simulink model "s_b4a4x32kf_nb"  (R2018a)
settings: Solver=VariableStepDiscrete  StartTime=0.0  StopTime=10000  RelTol=1e-3
undefined symbols (not defined in the file): fft_stages, n_bits_ants, n_bits_xengs
libraries: xbsIndex_r4 x21193, casper_library_misc x37, casper_library_scopes x13, casper_library_delays x8, xbsReplacements_r4 x6, xps_library x4
(part 98 of 274)

== system s_b4a4x32kf_nb/sys2/pkt_reord/Subsystem7 ==
  dv : Inport
  Constant8 : xbsIndex_r4/Constant  const=clk_rate  gui_display_data_type=Fixed-point  arith_type=Unsigned  n_bits=ceil(log2(clk_rate))  bin_pt=0  preci_type=Single  exp_width=8  frac_width=24  explicit_period=on  period=1  equ=P=C  opselect=C  inp2=PCIN>>17  opr=+  inp1=P  carry=CIN  dbl_ovrd=off  block_type=constant
      settings: SourceProductName=The database /home/jmanley/.matlab/R2018a/slblocks_master.db is locked, or a table in the database is locked. (database is locked)  block_version=11.4
  Counter1 : xbsIndex_r4/Counter  cnt_type=Count Limited  cnt_to=clk_rate  operation=Up  start_count=0  cnt_by_val=1  arith_type=Unsigned  n_bits=ceil(log2(clk_rate))  bin_pt=0  load_pin=off  rst=off  en=off  explicit_period=on  period=1  use_behavioral_HDL=off  implementation=Fabric  dbl_ovrd=off  block_type=counter
      settings: SourceProductName=The database /home/jmanley/.matlab/R2018a/slblocks_master.db is locked, or a table in the database is locked. (database is locked)
  Counter6 : xbsIndex_r4/Counter  cnt_type=Free Running  cnt_to=Inf  operation=Up  start_count=0  cnt_by_val=1  arith_type=Unsigned  n_bits=32  bin_pt=0  load_pin=off  rst=on  en=on  explicit_period=on  period=1  use_behavioral_HDL=off  implementation=Fabric  dbl_ovrd=off  block_type=counter
      settings: SourceProductName=The database /home/jmanley/.matlab/R2018a/slblocks_master.db is locked, or a table in the database is locked. (database is locked)
  Delay : xbsIndex_r4/Delay  rst=off  infoeditControl=Selection of Reset will increase slice count due to use of real FFs and instead of SRLs  en=on  latency=1  reg_retiming=on  dbl_ovrd=off  block_type=delay
      settings: SourceProductName=The database /home/jmanley/.matlab/R2018a/slblocks_master.db is locked, or a table in the database is locked. (database is locked)  infoedit=Hardware notes: A delay line is a chain, each link of which is an SRL16 or SRL32 followed by a flip-flop.
  Delay5 : xbsIndex_r4/Delay  rst=off  infoeditControl=Selection of Reset will increase slice count due to use of real FFs and instead of SRLs  en=off  latency=1  reg_retiming=on  dbl_ovrd=off  block_type=delay
      settings: SourceProductName=The database /home/jmanley/.matlab/R2018a/slblocks_master.db is locked, or a table in the database is locked. (database is locked)  infoedit=Hardware notes: A delay line is a chain, each link of which is an SRL16 or SRL32 followed by a flip-flop.
  Relational : xbsIndex_r4/Relational  mode=a=b  op_type=Bool  en=off  latency=1  dbl_ovrd=off  block_type=relational
      settings: SourceProductName=The database /home/jmanley/.matlab/R2018a/slblocks_master.db is locked, or a table in the database is locked. (database is locked)
  per_sec : Outport
  wires:
  Delay/1 -> per_sec/1
  Counter6/1 -> Delay/1
  dv/1 -> Delay5/1
  Relational/1 -> Delay/2, Counter6/1
  Counter1/1 -> Relational/1
  Delay5/1 -> Counter6/2
  Constant8/1 -> Relational/2

== system s_b4a4x32kf_nb/sys2/pkt_reord/bus_expand ==
  bus_in : Inport
  reinterpret1 : xbsIndex_r4/Reinterpret  force_arith_type=on  arith_type=Unsigned  force_bin_pt=on  bin_pt=0  block_type=reinterpret
      settings: SourceProductName=The database /home/jmanley/.matlab/R2018a/slblocks_master.db is locked, or a table in the database is locked. (database is locked)
  slice1 : xbsIndex_r4/Slice  nbits=32  boolean_output=off  mode=Upper Bit Location + Width  bit1=-1  base1=MSB of Input  bit0=0  base0=LSB of Input  dbl_ovrd=off  block_type=slice
      settings: SourceProductName=The database /home/jmanley/.matlab/R2018a/slblocks_master.db is locked, or a table in the database is locked. (database is locked)
  slice2 : xbsIndex_r4/Slice  nbits=1  boolean_output=on  mode=Upper Bit Location + Width  bit1=0  base1=MSB of Input  bit0=0  base0=LSB of Input  dbl_ovrd=off  block_type=slice
      settings: SourceProductName=The database /home/jmanley/.matlab/R2018a/slblocks_master.db is locked, or a table in the database is locked. (database is locked)
  msb_out2 : Outport
  lsb_out1 : Outport  Port=2
  wires:
  bus_in/1 -> slice2/1, slice1/1
  slice2/1 -> msb_out2/1
  slice1/1 -> reinterpret1/1
  reinterpret1/1 -> lsb_out1/1

== system s_b4a4x32kf_nb/sys2/pkt_reord/bus_replicate ==
  in : Inport
  bussify : Subsystem  mask(bus_create){inputNum=1}
      mask prompts: inputNum "Number of inputs:"
      mask init:
      | bus_create_init(gcb,...
      |     'inputNum', inputNum);
  out : Outport
  wires:
  in/1 -> bussify/1(in1)
  bussify/1(bus_out) -> out/1

== system s_b4a4x32kf_nb/sys2/pkt_reord/input_control ==
  note: Allow writing to windows
      | up to 1/2 the total buffer size
      |  behind the current maximum
      | mcnt
  data_in : Inport
  valid : Inport  Port=2
  pkt_idx : Inport  Port=3
  time_freq : Inport  Port=4
  src : Inport  Port=5
  pkt_size : Inport  Port=6
  n_src : Inport  Port=7
  AddSub2 : xbsIndex_r4/AddSub  mode=Addition  use_carryin=off  use_carryout=off  en=off  latency=2  precision=User Defined  arith_type=Unsigned  n_bits=n_bits_timestamp+chan_bits-xeng_bits  bin_pt=0  quantization=Truncate  overflow=Wrap  use_behavioral_HDL=on  hw_selection=Fabric  pipelined=off  use_rpm=on  dbl_ovrd=off  block_type=addsub
      settings: SourceProductName=The database /home/jmanley/.matlab/R2018a/slblocks_master.db is locked, or a table in the database is locked. (database is locked)  xl_area=[0, 0, 0, 0, 0, 0, 0]  block_version=10.1.3
  Constant2 : xbsIndex_r4/Constant  const=2^(window_bits - 1)  gui_display_data_type=Fixed-point  arith_type=Unsigned  n_bits=n_bits_timestamp+chan_bits-xeng_bits  bin_pt=0  preci_type=Single  exp_width=8  frac_width=24  explicit_period=on  period=1  equ=P=C  opselect=C  inp2=PCIN>>17  opr=+  inp1=P  carry=CIN  dbl_ovrd=off  block_type=constant
      settings: SourceProductName=The database /home/jmanley/.matlab/R2018a/slblocks_master.db is locked, or a table in the database is locked. (database is locked)
  Constant4 : xbsIndex_r4/Constant  const=0  gui_display_data_type=Boolean  arith_type=Boolean  n_bits=16  bin_pt=14  preci_type=Single  exp_width=8  frac_width=24  explicit_period=on  period=1  equ=P=C  opselect=C  inp2=PCIN>>17  opr=+  inp1=P  carry=CIN  dbl_ovrd=off  block_type=constant
      settings: SourceProductName=The database /home/jmanley/.matlab/R2018a/slblocks_master.db is locked, or a table in the database is locked. (database is locked)  block_version=11.4
  Delay{11,13..14,16} (4 alike) : xbsIndex_r4/Delay  rst=off  infoeditControl=Selection of Reset will increase slice count due to use of real FFs and instead of SRLs  en=off  latency=1  reg_retiming=on  dbl_ovrd=off  block_type=delay
      settings: SourceProductName=The database /home/jmanley/.matlab/R2018a/slblocks_master.db is locked, or a table in the database is locked. (database is locked)  infoedit=Hardware notes: A delay line is a chain, each link of which is an SRL16 or SRL32 followed by a flip-flop.  xl_area=[0, 0, 0, 0, 0, 0, 0]
  Delay{2,4..5,8..9} (5 alike) : xbsIndex_r4/Delay  rst=off  infoeditControl=Selection of Reset will increase slice count due to use of real FFs and instead of SRLs  en=off  latency=2  reg_retiming=on  dbl_ovrd=off  block_type=delay
      settings: SourceProductName=The database /home/jmanley/.matlab/R2018a/slblocks_master.db is locked, or a table in the database is locked. (database is locked)  xl_area=[0, 0, 0, 0, 0, 0, 0]
  Delay{3,21,24..27} (6 alike) : xbsIndex_r4/Delay  rst=off  infoeditControl=Selection of Reset will increase slice count due to use of real FFs and instead of SRLs  en=off  latency=3  reg_retiming=on  dbl_ovrd=off  block_type=delay
      settings: SourceProductName=The database /home/jmanley/.matlab/R2018a/slblocks_master.db is locked, or a table in the database is locked. (database is locked)  xl_area=[0, 0, 0, 0, 0, 0, 0]
  Delay23 : xbsIndex_r4/Delay  rst=off  infoeditControl=Selection of Reset will increase slice count due to use of real FFs and instead of SRLs  en=off  latency=4  reg_retiming=on  dbl_ovrd=off  block_type=delay
      settings: SourceProductName=The database /home/jmanley/.matlab/R2018a/slblocks_master.db is locked, or a table in the database is locked. (database is locked)  xl_area=[0, 0, 0, 0, 0, 0, 0]
  Inverter : xbsIndex_r4/Inverter  en=off  latency=0  dbl_ovrd=off  block_type=inv
      settings: SourceProductName=The database /home/jmanley/.matlab/R2018a/slblocks_master.db is locked, or a table in the database is locked. (database is locked)
  Logical : xbsIndex_r4/Logical  logical_function=AND  inputs=3  en=off  latency=1  precision=Full  arith_type=Unsigned  n_bits=8  bin_pt=2  align_bp=on  dbl_ovrd=off  block_type=logical
      settings: SourceProductName=The database /home/jmanley/.matlab/R2018a/slblocks_master.db is locked, or a table in the database is locked. (database is locked)  xl_area=[0, 0, 0, 0, 0, 0, 0]
  Logical1 : xbsIndex_r4/Logical  logical_function=AND  inputs=2  en=off  latency=0  precision=Full  arith_type=Unsigned  n_bits=8  bin_pt=2  align_bp=on  dbl_ovrd=off  block_type=logical
      settings: SourceProductName=The database /home/jmanley/.matlab/R2018a/slblocks_master.db is locked, or a table in the database is locked. (database is locked)  xl_area=[0, 0, 0, 0, 0, 0, 0]
  Mult : xbsIndex_r4/Mult  precision=Full  arith_type=Unsigned  n_bits=buf_bits  bin_pt=0  quantization=Truncate  overflow=Wrap  en=off  latency=3  use_behavioral_HDL=off  opt=Speed  use_embedded=on  optimum_pipeline=off  pipeline=on  dbl_ovrd=off  use_rpm=on  placement_style=Triangular  block_type=mult
      settings: SourceProductName=The database /home/jmanley/.matlab/R2018a/slblocks_master.db is locked, or a table in the database is locked. (database is locked)
  Mult1 : xbsIndex_r4/Mult  precision=Full  arith_type=Unsigned  n_bits=buf_bits  bin_pt=0  quantization=Truncate  overflow=Wrap  en=off  latency=3  use_behavioral_HDL=off  opt=Speed  use_embedded=on  optimum_pipeline=off  pipeline=on  dbl_ovrd=off  use_rpm=on  placement_style=Triangular  block_type=mult
      settings: SourceProductName=The database /home/jmanley/.matlab/R2018a/slblocks_master.db is locked, or a table in the database is locked. (database is locked)
  Relational : xbsIndex_r4/Relational  mode=a>=b  op_type=Bool  en=off  latency=2  dbl_ovrd=off  block_type=relational
      settings: SourceProductName=The database /home/jmanley/.matlab/R2018a/slblocks_master.db is locked, or a table in the database is locked. (database is locked)  xl_area=[0, 0, 0, 0, 0, 0, 0]  block_version=10.1.3
  Relational2 : xbsIndex_r4/Relational  mode=a<b  op_type=Bool  en=off  latency=2  dbl_ovrd=off  block_type=relational
      settings: SourceProductName=The database /home/jmanley/.matlab/R2018a/slblocks_master.db is locked, or a table in the database is locked. (database is locked)  xl_area=[0, 0, 0, 0, 0, 0, 0]  block_version=10.1.3
  Slice1 : xbsIndex_r4/Slice  nbits=buf_bits  boolean_output=off  mode=Lower Bit Location + Width  bit1=0  base1=MSB of Input  bit0=0  base0=LSB of Input  dbl_ovrd=off  block_type=slice
      settings: SourceProductName=The database /home/jmanley/.matlab/R2018a/slblocks_master.db is locked, or a table in the database is locked. (database is locked)
  Slice2 : xbsIndex_r4/Slice  nbits=window_bits  boolean_output=off  mode=Lower Bit Location + Width  bit1=0  base1=MSB of Input  bit0=0  base0=LSB of Input  dbl_ovrd=off  block_type=slice
      settings: SourceProductName=The database /home/jmanley/.matlab/R2018a/slblocks_master.db is locked, or a table in the database is locked. (database is locked)
  Terminator : Terminator
  adder_tree : Subsystem  Tag=cmac_delinked  mask(adder_tree){n_inputs=3, csp_latency=2, adder_imp=Fabric, first_stage_hdl=off, floating_point=off, float_type=single, frac_width=0, exp_width=0}
      mask prompts: n_inputs "Number of Inputs"; csp_latency "Add Latency"; adder_imp "Adder implementation"; first_stage_hdl "Use behavioural HDL for first stage of adders"; floating_point "floating point"; float_type "float type"; frac_width "fraction length"; exp_width "exponent length"
      mask help:
      | Sums all inputs using a tree of adds and delays.
      |
      | Number of inputs: The number of inputs to the block to be summed
      | Add latency: The number of clock cycles to perform one addition (affects timing)..
      | Adder implementation: choice of fabric or DSP48E core, or behavioral HDL
      | Use behavioural HDL for first stage of adders: Causes the first stage of adders to be absorbed into DSP blocks if multipliers precede them (Virtex 5). Overrides Adder implementation
      mask init: same as s_b4a4x32kf_nb/sys0/pkt_reord/input_control/adder_tree
      settings: AttributesFormatString=latency 4
      mask Help: eval('xlWeb(''http://casper.berkeley.edu/wiki/Adder_tree'')')
      mask TypeOptions adder_imp: Behavioral | Fabric | DSP48
      mask Callback floating_point:
      | onoff = get_param(gcb, 'floating_point');
      | if strcmp(onoff,'on')
      |     enable_fixpt = 'off'
      |     set_param_state(gcb, 'float_type', 'on')
      | 
      |     f_type = get_param(gcb, 'float_type')
      |     if strcmp(f_type,'custom')
      |         set_param_state(gcb, 'exp_width', 'on')
      |         set_param_state(gcb, 'frac_width', 'on')
      |     else
      |         set_param_state(gcb, 'exp_width', 'off')
      |         set_param_state(gcb, 'frac_width', 'off')
      |     end
      | 
      | 
      | else
      |     enable_fixpt = 'on'
      |     set_param_state(gcb, 'float_type', 'off')
      |     set_param_state(gcb, 'exp_width', 'off')
      |     set_param_state(gcb, 'frac_width', 'off')
      | end
      mask TypeOptions float_type: single | custom
      mask Callback float_type:
      | f_type = get_param(gcb, 'float_type')
      | if strcmp(f_type,'custom')
      |     set_param_state(gcb, 'exp_width', 'on')
      |     set_param_state(gcb, 'frac_width', 'on')
      | else
      |     set_param_state(gcb, 'exp_width', 'off')
      |     set_param_state(gcb, 'frac_width', 'off')
      | end
  freq_window : xbsIndex_r4/Mult  precision=Full  arith_type="Signed  (2's comp)"  n_bits=16  bin_pt=14  quantization=Truncate  overflow=Wrap  en=off  latency=3  use_behavioral_HDL=off  opt=Speed  use_embedded=on  optimum_pipeline=off  pipeline=on  dbl_ovrd=off  use_rpm=on  placement_style=Triangular  block_type=mult
      settings: SourceProductName=The database /home/jmanley/.matlab/R2018a/slblocks_master.db is locked, or a table in the database is locked. (database is locked)
  mcnt_thresh : Subsystem
  maxcnt : Outport
  wr_addr : Outport  Port=2
  wr_data : Outport  Port=3
  we : Outport  Port=4
  discarding : Outport  Port=5
  mcnt_timeout : Outport  Port=6
  wires:
  Constant2/1 -> AddSub2/2
  Delay2/1 -> Delay4/1
  Delay3/1 -> Delay2/1, [data_add]
  data_in/1 -> Delay3/1
  adder_tree/2(dout) -> Slice1/1
  Slice2/1 -> Mult1/2
  freq_window/1 -> Mult1/1
  n_src/1 -> freq_window/1
  Mult1/1 -> adder_tree/2(din1), [brds_pkt_size_time]
  Delay27/1 -> AddSub2/1
  Delay26/1 -> mcnt_thresh/1(mcnt)
  Delay25/1 -> Delay5/1
  Constant4/1 -> adder_tree/1(sync)
  Mult/1 -> adder_tree/3(din2), [src_pkt_size]
  Delay21/1 -> [pkt_idx], adder_tree/4(din3)
  time_freq/1 -> Slice2/1, Delay26/1, Delay25/1, [mcnt_in], Delay27/1
  Delay24/1 -> mcnt_thresh/2(en), [valid_add], Delay23/1
  src/1 -> Mult/1
  pkt_size/1 -> freq_window/2, Mult/2
  pkt_idx/1 -> Delay21/1
  valid/1 -> Delay24/1
  Delay9/1 -> Delay13/1
  Slice1/1 -> Delay16/1
  Delay4/1 -> Delay11/1
  Delay23/1 -> Logical/3, Delay14/1
  Logical/1 -> Inverter/1, [we], we/1
  Relational/1 -> Logical/2
  Delay5/1 -> Relational/2
  mcnt_thresh/1(maxcnt) -> Delay9/1, Relational2/1, Relational/1
  Relational2/1 -> Logical/1
  adder_tree/1(sync_out) -> Terminator/1
  Logical1/1 -> [discarding], discarding/1
  Inverter/1 -> Logical1/1
  mcnt_thresh/2(mcnt_timeout) -> [timeout], Delay8/1
  AddSub2/1 -> Relational2/2
  Delay11/1 -> wr_data/1, [wr_data]
  Delay13/1 -> maxcnt/1, [max_mcnt]
  Delay14/1 -> Logical1/2
  Delay8/1 -> mcnt_timeout/1
  Delay16/1 -> [wr_addr], wr_addr/1

== system s_b4a4x32kf_nb/sys2/pkt_reord/munge ==
  din : Inport
  join : Subsystem  mask(bus_create){inputNum=16}
      mask prompts: inputNum "Number of inputs:"
      mask init:
      | bus_create_init(gcb,...
      |     'inputNum', inputNum);
  reinterpret : xbsIndex_r4/Reinterpret  force_arith_type=on  arith_type=Unsigned  force_bin_pt=on  bin_pt=0  block_type=reinterpret
      settings: SourceProductName=The database /home/jmanley/.matlab/R2018a/slblocks_master.db is locked, or a table in the database is locked. (database is locked)
  reinterpret_out : xbsIndex_r4/Reinterpret  force_arith_type=on  arith_type=Unsigned  force_bin_pt=on  bin_pt=0  block_type=reinterpret
      settings: SourceProductName=The database /home/jmanley/.matlab/R2018a/slblocks_master.db is locked, or a table in the database is locked. (database is locked)
  split : Subsystem  mask(bus_expand){mode=divisions of arbitrary size, outputNum=1, outputWidth=[1 32 32 32 32 32 32 32 32], outputBinaryPt=[0 0 0 0 0 0 0 0 0], outputArithmeticType=[0 0 0 0 0 0 0 0 0], show_format=off, outputToWorkspace=off, variablePrefix=out, outputToModelAsWell=on}
      mask prompts: outputNum "Number of outputs:"; outputWidth "Output width [msb ... lsb]:"; outputBinaryPt "Output binary point position [msb ... lsb]:"; outputArithmeticType "Output arithmetic type (ufix=0, fix=1, bool=2) [msb ... lsb]:"; show_format "Print format string?"; outputToWorkspace "Output to workspace?"; variablePrefix "Variable name prefix:"; outputToModelAsWell "Output to model as well?"
      mask help:
      | Expands a 'bus' made using a bus_create or Xilinx
      | concat block.
      | The input will be divided into the specified number
      | of outputs with the specified arithmetic types.
      | Divisions are made from most significant bit.
      mask init: same as s_b4a4x32kf_nb/bus_expand
      settings: AttributesFormatString=9 outputs
      mask TypeOptions mode: divisions of equal size | divisions of arbitrary size
      mask Callback mode: bus_expand_callback();
      mask Callback outputWidth: bus_expand_callback();
      mask Callback outputToWorkspace: bus_expand_callback();
  dout : Outport
  wires:
  reinterpret_out/1 -> dout/1
  din/1 -> reinterpret/1
  reinterpret/1 -> split/1(bus_in)
  join/1(bus_out) -> reinterpret_out/1
  split/1(msb_out9) -> join/1(in1), join/3(in3), join/5(in5), join/7(in7), join/9(in9), join/11(in11), join/13(in13), join/15(in15)
  split/9(lsb_out1) -> join/2(in2)
  split/8(out2) -> join/4(in4)
  split/7(out3) -> join/6(in6)
  split/6(out4) -> join/8(in8)
  split/5(out5) -> join/10(in10)
  split/4(out6) -> join/12(in12)
  split/3(out7) -> join/14(in14)
  split/2(out8) -> join/16(in16)

== system s_b4a4x32kf_nb/sys2/pkt_reord/munge1 ==
  din : Inport
  join : Subsystem  mask(bus_create){inputNum=2}
      mask prompts: inputNum "Number of inputs:"
      mask init:
      | bus_create_init(gcb,...
      |     'inputNum', inputNum);
  reinterpret : xbsIndex_r4/Reinterpret  force_arith_type=on  arith_type=Unsigned  force_bin_pt=on  bin_pt=0  block_type=reinterpret
      settings: SourceProductName=The database /home/jmanley/.matlab/R2018a/slblocks_master.db is locked, or a table in the database is locked. (database is locked)
  reinterpret_out : xbsIndex_r4/Reinterpret  force_arith_type=on  arith_type=Unsigned  force_bin_pt=on  bin_pt=0  block_type=reinterpret
      settings: SourceProductName=The database /home/jmanley/.matlab/R2018a/slblocks_master.db is locked, or a table in the database is locked. (database is locked)
  split : Subsystem  mask(bus_expand){mode=divisions of arbitrary size, outputNum=1, outputWidth=[1 32], outputBinaryPt=[0 0], outputArithmeticType=[0 0], show_format=off, outputToWorkspace=off, variablePrefix=out, outputToModelAsWell=on}
      mask prompts: outputNum "Number of outputs:"; outputWidth "Output width [msb ... lsb]:"; outputBinaryPt "Output binary point position [msb ... lsb]:"; outputArithmeticType "Output arithmetic type (ufix=0, fix=1, bool=2) [msb ... lsb]:"; show_format "Print format string?"; outputToWorkspace "Output to workspace?"; variablePrefix "Variable name prefix:"; outputToModelAsWell "Output to model as well?"
      mask help:
      | Expands a 'bus' made using a bus_create or Xilinx
      | concat block.
      | The input will be divided into the specified number
      | of outputs with the specified arithmetic types.
      | Divisions are made from most significant bit.
      mask init: same as s_b4a4x32kf_nb/bus_expand
      settings: AttributesFormatString=2 outputs
      mask TypeOptions mode: divisions of equal size | divisions of arbitrary size
      mask Callback mode: bus_expand_callback();
      mask Callback outputWidth: bus_expand_callback();
      mask Callback outputToWorkspace: bus_expand_callback();
  dout : Outport
  wires:
  reinterpret_out/1 -> dout/1
  din/1 -> reinterpret/1
  reinterpret/1 -> split/1(bus_in)
  join/1(bus_out) -> reinterpret_out/1
  split/1(msb_out2) -> join/1(in1)
  split/2(lsb_out1) -> join/2(in2)

== system s_b4a4x32kf_nb/sys2/pkt_reord/output_control ==
  note: add delay here
      | to ensure mcnt has had
      | chance to calculate
      | correctly
  note: If reading from addr 0 (corresponding to f=0,nant,2nant,...)
      | and max_mcnt (skipping window_bits for the difference
      | between max_mcnt and rd_mcnt) is 0 for sync_bits, then
      | issue a sync.
  note: If we need to ship a window,
      | send the data on a window edge
  note: Decide whether to ship
      | a window or not:
  note: If the read window is 1/2
      | the total buffer size (or more)
      | behind the write window,
      | it is time to ship it out.
  note: rd_addr is counting for
      | output words to
      | X engines
  maxcnt : Inport
  AddSub1 : xbsIndex_r4/AddSub  mode=Subtraction  use_carryin=off  use_carryout=off  en=off  latency=2  precision=User Defined  arith_type=Unsigned  n_bits=window_bits  bin_pt=0  quantization=Truncate  overflow=Wrap  use_behavioral_HDL=on  hw_selection=Fabric  pipelined=off  use_rpm=on  dbl_ovrd=off  block_type=addsub
      settings: SourceProductName=The database /home/jmanley/.matlab/R2018a/slblocks_master.db is locked, or a table in the database is locked. (database is locked)  xl_area=[0, 0, 0, 0, 0, 0, 0]  block_version=10.1.3
  Concat1 : xbsIndex_r4/Concat  num_inputs=2  dbl_ovrd=off  block_type=concat
      settings: SourceProductName=The database /home/jmanley/.matlab/R2018a/slblocks_master.db is locked, or a table in the database is locked. (database is locked)  block_version=10.1.3
  Concat2 : xbsIndex_r4/Concat  num_inputs=2  dbl_ovrd=off  block_type=concat
      settings: SourceProductName=The database /home/jmanley/.matlab/R2018a/slblocks_master.db is locked, or a table in the database is locked. (database is locked)  block_version=10.1.3
  Constant1 : xbsIndex_r4/Constant  const=2^(window_bits - 1)  gui_display_data_type=Fixed-point  arith_type=Unsigned  n_bits=window_bits  bin_pt=0  preci_type=Single  exp_width=8  frac_width=24  explicit_period=on  period=1  equ=P=C  opselect=C  inp2=PCIN>>17  opr=+  inp1=P  carry=CIN  dbl_ovrd=off  block_type=constant
      settings: SourceProductName=The database /home/jmanley/.matlab/R2018a/slblocks_master.db is locked, or a table in the database is locked. (database is locked)
  Constant3 : xbsIndex_r4/Constant  const=0  gui_display_data_type=Fixed-point  arith_type=Unsigned  n_bits=sync_bits - x_int_bits - ant_bits - window_bits  bin_pt=0  preci_type=Single  exp_width=8  frac_width=24  explicit_period=on  period=1  equ=P=C  opselect=C  inp2=PCIN>>17  opr=+  inp1=P  carry=CIN  dbl_ovrd=off  block_type=constant
      settings: SourceProductName=The database /home/jmanley/.matlab/R2018a/slblocks_master.db is locked, or a table in the database is locked. (database is locked)
  Delay1 : xbsIndex_r4/Delay  rst=off  infoeditControl=Selection of Reset will increase slice count due to use of real FFs and instead of SRLs  en=off  latency=1  reg_retiming=on  dbl_ovrd=off  block_type=delay
      settings: SourceProductName=The database /home/jmanley/.matlab/R2018a/slblocks_master.db is locked, or a table in the database is locked. (database is locked)  xl_area=[0, 0, 0, 0, 0, 0, 0]
  Delay3 : xbsIndex_r4/Delay  rst=off  infoeditControl=Selection of Reset will increase slice count due to use of real FFs and instead of SRLs  en=off  latency=2  reg_retiming=on  dbl_ovrd=off  block_type=delay
      settings: SourceProductName=The database /home/jmanley/.matlab/R2018a/slblocks_master.db is locked, or a table in the database is locked. (database is locked)  xl_area=[0, 0, 0, 0, 0, 0, 0]
  Delay6 : xbsIndex_r4/Delay  rst=off  infoeditControl=Selection of Reset will increase slice count due to use of real FFs and instead of SRLs  en=off  latency=1  reg_retiming=on  dbl_ovrd=off  block_type=delay
      settings: SourceProductName=The database /home/jmanley/.matlab/R2018a/slblocks_master.db is locked, or a table in the database is locked. (database is locked)  xl_area=[0, 0, 0, 0, 0, 0, 0]
  Delay7 : xbsIndex_r4/Delay  rst=off  infoeditControl=Selection of Reset will increase slice count due to use of real FFs and instead of SRLs  en=off  latency=2  reg_retiming=on  dbl_ovrd=off  block_type=delay
      settings: SourceProductName=The database /home/jmanley/.matlab/R2018a/slblocks_master.db is locked, or a table in the database is locked. (database is locked)  xl_area=[0, 0, 0, 0, 0, 0, 0]
  Gateway Out{1..18} (18 alike) : xbsIndex_r4/Gateway Out  inherit_from_input=off  hdl_port=off  rows=1  columns=1  UseAsDAC=off  DACChannel='1'  interface=None  automatic_assignment=on  address_offset=hex2dec('00')  intf_name=''  intf_description=''  timing_constraint=None  locs_specified=off  LOCs={}  io_standard={}  block_type=gatewayout
      settings: SourceProductName=The database /home/jmanley/.matlab/R2018a/slblocks_master.db is locked, or a table in the database is locked. (database is locked)  infoedit="Gateway out block.  Converts Xilinx fixed point inputs into ouputs of type Simulink integer, double, or fixed point.<P><P>Hardware notes:  In hardware these blocks become top level output ports or are discarded, depending on how they are configured."  xl_area=[0, 0, 0, 0, 0, 0, 0]  block_version=10.1.3
  Logical1 : xbsIndex_r4/Logical  logical_function=AND  inputs=2  en=off  latency=0  precision=Full  arith_type=Unsigned  n_bits=8  bin_pt=2  align_bp=on  dbl_ovrd=off  block_type=logical
      settings: SourceProductName=The database /home/jmanley/.matlab/R2018a/slblocks_master.db is locked, or a table in the database is locked. (database is locked)  xl_area=[0, 0, 0, 0, 0, 0, 0]
  Logical2 : xbsIndex_r4/Logical  logical_function=AND  inputs=2  en=off  latency=0  precision=Full  arith_type=Unsigned  n_bits=8  bin_pt=2  align_bp=on  dbl_ovrd=off  block_type=logical
      settings: SourceProductName=The database /home/jmanley/.matlab/R2018a/slblocks_master.db is locked, or a table in the database is locked. (database is locked)  xl_area=[0, 0, 0, 0, 0, 0, 0]
  Logical4 : xbsIndex_r4/Logical  logical_function=AND  inputs=2  en=off  latency=0  precision=Full  arith_type=Unsigned  n_bits=8  bin_pt=2  align_bp=on  dbl_ovrd=off  block_type=logical
      settings: SourceProductName=The database /home/jmanley/.matlab/R2018a/slblocks_master.db is locked, or a table in the database is locked. (database is locked)  xl_area=[0, 0, 0, 0, 0, 0, 0]
  Register : xbsIndex_r4/Register  init=0  rst=off  en=on  dbl_ovrd=off  block_type=register
      settings: SourceProductName=The database /home/jmanley/.matlab/R2018a/slblocks_master.db is locked, or a table in the database is locked. (database is locked)
  Register1 : xbsIndex_r4/Register  init=0  rst=off  en=on  dbl_ovrd=off  block_type=register
      settings: SourceProductName=The database /home/jmanley/.matlab/R2018a/slblocks_master.db is locked, or a table in the database is locked. (database is locked)
  Register3 : xbsIndex_r4/Register  init=0  rst=off  en=on  dbl_ovrd=off  block_type=register
      settings: SourceProductName=The database /home/jmanley/.matlab/R2018a/slblocks_master.db is locked, or a table in the database is locked. (database is locked)
  Relational1 : xbsIndex_r4/Relational  mode=a>=b  op_type=Bool  en=off  latency=1  dbl_ovrd=off  block_type=relational
      settings: SourceProductName=The database /home/jmanley/.matlab/R2018a/slblocks_master.db is locked, or a table in the database is locked. (database is locked)  xl_area=[0, 0, 0, 0, 0, 0, 0]  block_version=10.1.3
  Relational4 : xbsIndex_r4/Relational  mode=a=b  op_type=Bool  en=off  latency=1  dbl_ovrd=off  block_type=relational
      settings: SourceProductName=The database /home/jmanley/.matlab/R2018a/slblocks_master.db is locked, or a table in the database is locked. (database is locked)  xl_area=[0, 0, 0, 0, 0, 0, 0]  block_version=10.1.3
  Slice1 : xbsIndex_r4/Slice  nbits=window_bits  boolean_output=off  mode=Lower Bit Location + Width  bit1=0  base1=MSB of Input  bit0=0  base0=LSB of Input  dbl_ovrd=off  block_type=slice
      settings: SourceProductName=The database /home/jmanley/.matlab/R2018a/slblocks_master.db is locked, or a table in the database is locked. (database is locked)  infoedit="Extracts a given range of bits from each input sample and presents it at the output.  The output type is ordinarily unsigned with binary point at zero, but can be Boolean when the slice is one bit wide.<P><P>Hardware notes: In hardware this block costs nothing."  block_version=10.1.3
  Slice2 : xbsIndex_r4/Slice  nbits=1  boolean_output=on  mode=Upper Bit Location + Width  bit1=0  base1=MSB of Input  bit0=0  base0=LSB of Input  dbl_ovrd=off  block_type=slice
      settings: SourceProductName=The database /home/jmanley/.matlab/R2018a/slblocks_master.db is locked, or a table in the database is locked. (database is locked)  infoedit="Extracts a given range of bits from each input sample and presents it at the output.  The output type is ordinarily unsigned with binary point at zero, but can be Boolean when the slice is one bit wide.<P><P>Hardware notes: In hardware this block costs nothing."  block_version=10.1.3
  Slice3 : xbsIndex_r4/Slice  nbits=window_bits  boolean_output=off  mode=Lower Bit Location + Width  bit1=0  base1=MSB of Input  bit0=0  base0=LSB of Input  dbl_ovrd=off  block_type=slice
      settings: SourceProductName=The database /home/jmanley/.matlab/R2018a/slblocks_master.db is locked, or a table in the database is locked. (database is locked)  infoedit="Extracts a given range of bits from each input sample and presents it at the output.  The output type is ordinarily unsigned with binary point at zero, but can be Boolean when the slice is one bit wide.<P><P>Hardware notes: In hardware this block costs nothing."  block_version=10.1.3
  Slice4 : xbsIndex_r4/Slice  nbits=x_int_bits + ant_bits - n_bits_output_words  boolean_output=off  mode=Lower Bit Location + Width  bit1=0  base1=MSB of Input  bit0=0  base0=LSB of Input  dbl_ovrd=off  block_type=slice
      settings: SourceProductName=The database /home/jmanley/.matlab/R2018a/slblocks_master.db is locked, or a table in the database is locked. (database is locked)  block_version=10.1.3
  Slice5 : xbsIndex_r4/Slice  nbits=window_bits  boolean_output=off  mode=Two Bit Locations  bit1=sync_bits - x_int_bits - ant_bits - 1  base1=LSB of Input  bit0=window_bits  base0=LSB of Input  dbl_ovrd=off  block_type=slice
      settings: SourceProductName=The database /home/jmanley/.matlab/R2018a/slblocks_master.db is locked, or a table in the database is locked. (database is locked)  infoedit="Extracts a given range of bits from each input sample and presents it at the output.  The output type is ordinarily unsigned with binary point at zero, but can be Boolean when the slice is one bit wide.<P><P>Hardware notes: In hardware this block costs nothing."  block_version=10.1.3
  Slice6 : xbsIndex_r4/Slice  nbits=1  boolean_output=on  mode=Upper Bit Location + Width  bit1=0  base1=MSB of Input  bit0=0  base0=LSB of Input  dbl_ovrd=off  block_type=slice
      settings: SourceProductName=The database /home/jmanley/.matlab/R2018a/slblocks_master.db is locked, or a table in the database is locked. (database is locked)  infoedit="Extracts a given range of bits from each input sample and presents it at the output.  The output type is ordinarily unsigned with binary point at zero, but can be Boolean when the slice is one bit wide.<P><P>Hardware notes: In hardware this block costs nothing."  block_version=10.1.3
  Slice7 : xbsIndex_r4/Slice  nbits=1  boolean_output=off  mode=Two Bit Locations  bit1=0  base1=MSB of Input  bit0=window_bits  base0=LSB of Input  dbl_ovrd=off  block_type=slice
      settings: SourceProductName=The database /home/jmanley/.matlab/R2018a/slblocks_master.db is locked, or a table in the database is locked. (database is locked)  infoedit="Extracts a given range of bits from each input sample and presents it at the output.  The output type is ordinarily unsigned with binary point at zero, but can be Boolean when the slice is one bit wide.<P><P>Hardware notes: In hardware this block costs nothing."  block_version=10.1.3
  edge_detect : Subsystem  mask(edge_detect){edge=Both, polarity=Active High, x_in=[0 0.08 0.08 0.16 0.16 0.24 0.24 0.32 0.32 0.4], y_in=[-1 -1  1  1  1  1  1  1  1  1], x_out=[0.6 0.68 0.68 0.76 0.76 0.84 0.84 0.92 0.92 1], y_out=[-1 -1  1  1 -1 -1 -1 -1 -1 -1]}
      mask prompts: edge "Edge Type"; polarity "Output Polarity"; x_in "Input X Positions"; y_in "Input Y Positions"; x_out "Output X Positions"; y_out "Output Y Positions"
      mask help: Output is active for one-cycle after each edge of the specified type (i.e. rising, falling or both).
      mask init: same as s_b4a4x32kf_nb/edge_detect
      settings: AttributesFormatString=|
      | both edges
      | active high
      mask Help: Output is active for one-cycle after each edge of the specified type (i.e. rising, falling, or both).  Latency is zero.
      mask TypeOptions edge: Rising | Falling | Both
      mask TypeOptions polarity: Active High | Active Low
      mask Display:
      | plot(x_in_num,0.5+y_in_num*0.2);
      | plot(x_out_num,0.5+y_out_num*0.2);
  edge_detect1 : Subsystem  mask(edge_detect){edge=Both, polarity=Active High, x_in=[0 0.08 0.08 0.16 0.16 0.24 0.24 0.32 0.32 0.4], y_in=[-1 -1  1  1  1  1  1  1  1  1], x_out=[0.6 0.68 0.68 0.76 0.76 0.84 0.84 0.92 0.92 1], y_out=[-1 -1  1  1 -1 -1 -1 -1 -1 -1]}
      mask prompts: edge "Edge Type"; polarity "Output Polarity"; x_in "Input X Positions"; y_in "Input Y Positions"; x_out "Output X Positions"; y_out "Output Y Positions"
      mask help: Output is active for one-cycle after each edge of the specified type (i.e. rising, falling or both).
      mask init: same as s_b4a4x32kf_nb/edge_detect
      settings: AttributesFormatString=|
      | both edges
      | active high
      mask Help: Output is active for one-cycle after each edge of the specified type (i.e. rising, falling, or both).  Latency is zero.
      mask TypeOptions edge: Rising | Falling | Both
      mask TypeOptions polarity: Active High | Active Low
      mask Display:
      | plot(x_in_num,0.5+y_in_num*0.2);
      | plot(x_out_num,0.5+y_out_num*0.2);
  internal_descr_Scope : Scope  NumInputPorts=8
  internal_descr_Scope1 : Scope  NumInputPorts=10
  pulse_ext : Subsystem  mask(pulse_ext){pulse_len=2^(x_int_bits + ant_bits - n_bits_output_words)}
      mask prompts: pulse_len "Length of Pulse"
      mask help:
      | Extends a boolean signal to be high for the specified number of clocks after
      | the last high input.
      mask init:
      | bits = ceil(log2(pulse_len+1));
      mask Help: eval('xlWeb([getenv(''MLIB_ROOT''), ''\doc\htmlblocks\sp_pulse_ext\sp_pulse_ext.html''])')
  win_addr_cnt : xbsIndex_r4/Counter  cnt_type=Free Running  cnt_to=Inf  operation=Up  start_count=0  cnt_by_val=1  arith_type=Unsigned  n_bits=x_int_bits + ant_bits + 1 - n_bits_output_words  bin_pt=0  load_pin=off  rst=off  en=off  explicit_period=on  period=1  use_behavioral_HDL=off  implementation=Fabric  use_rpm=on  dbl_ovrd=off  block_type=counter
      settings: SourceProductName=The database /home/jmanley/.matlab/R2018a/slblocks_master.db is locked, or a table in the database is locked. (database is locked)  xl_area=[0, 0, 0, 0, 0, 0, 0]
  win_cnt : xbsIndex_r4/Counter  cnt_type=Free Running  cnt_to=Inf  operation=Up  start_count=0  cnt_by_val=1  arith_type=Unsigned  n_bits=window_bits + 1  bin_pt=0  load_pin=off  rst=off  en=on  explicit_period=off  period=1  use_behavioral_HDL=off  implementation=Fabric  use_rpm=on  dbl_ovrd=off  block_type=counter
      settings: SourceProductName=The database /home/jmanley/.matlab/R2018a/slblocks_master.db is locked, or a table in the database is locked. (database is locked)  xl_area=[0, 0, 0, 0, 0, 0, 0]
  gen_sync : Outport
  rd_en : Outport  Port=2
  rd_addr : Outport  Port=3
  rd_timefreq : Outport  Port=4
  wires:
  [current_window_out] -> Concat1/1
  [buffer_edge] -> [mcnt_sample], Register/2
  Gateway Out18/1 -> internal_descr_Scope1/10
  [sampled_mcnt] -> Gateway Out18/1
  Register/1 -> Concat2/1, [sampled_mcnt]
  Slice7/1 -> Register/1
  [maxcnt] -> Slice7/1, [offset_mcnt]
  Delay3/1 -> Logical1/2
  Gateway Out17/1 -> internal_descr_Scope1/9
  [mcnt_sample] -> Gateway Out17/1
  [rd_addr] -> Gateway Out2/1
  [rd_en] -> Gateway Out1/1
  [rd_addr] -> Gateway Out14/1
  [rd_en] -> Gateway Out9/1
  [rd_mcnt] -> Gateway Out13/1
  [ship_next_window] -> Gateway Out8/1
  [offset_mcnt] -> Gateway Out12/1
  [maxcnt] -> Gateway Out10/1
  [current_window_out] -> Gateway Out11/1
  Delay1/1 -> [current_window_out]
  win_cnt/1 -> Register1/1
  Delay6/1 -> Logical4/1
  Register3/1 -> Logical4/2
  pulse_ext/1(out) -> Delay6/1
  Logical4/1 -> [rd_en], rd_en/1
  [rd_mcnt] -> Gateway Out7/1
  Logical2/1 -> [gen_sync], gen_sync/1
  Gateway Out16/1 -> internal_descr_Scope/8
  [gen_sync] -> Gateway Out16/1
  [gen_sync] -> Gateway Out15/1
  Gateway Out15/1 -> internal_descr_Scope1/8
  Gateway Out14/1 -> internal_descr_Scope1/7
  Gateway Out9/1 -> internal_descr_Scope1/6
  Gateway Out8/1 -> internal_descr_Scope1/5
  Gateway Out13/1 -> internal_descr_Scope1/4
  Gateway Out12/1 -> internal_descr_Scope1/3
  Gateway Out11/1 -> internal_descr_Scope1/1
  Gateway Out10/1 -> internal_descr_Scope1/2
  [current_window_out] -> Concat2/2
  Gateway Out7/1 -> internal_descr_Scope/7
  [ship_window_now] -> Gateway Out6/1
  Gateway Out2/1 -> internal_descr_Scope/6
  Gateway Out1/1 -> internal_descr_Scope/5
  Gateway Out6/1 -> internal_descr_Scope/4
  [ship_next_window] -> Gateway Out5/1
  [current_window_out] -> Gateway Out3/1
  [maxcnt] -> Gateway Out4/1
  Gateway Out5/1 -> internal_descr_Scope/3
  Gateway Out4/1 -> internal_descr_Scope/1
  Gateway Out3/1 -> internal_descr_Scope/2
  Relational4/1 -> Logical2/2
  [ship_window_now] -> Register1/2, win_cnt/1
  Relational1/1 -> [ship_next_window]
  [maxcnt] -> Slice3/1
  [current_window] -> AddSub1/2
  Constant1/1 -> Relational1/2
  AddSub1/1 -> Relational1/1
  Slice3/1 -> AddSub1/1
  [ship_next_window] -> Delay3/1
  maxcnt/1 -> Slice5/1, [maxcnt]
  Register1/1 -> Slice2/1, Slice1/1
  Logical1/1 -> [ship_window_now], pulse_ext/1(in), Register3/2, Register3/1
  edge_detect/1(out) -> [buffer_edge], Logical2/1
  Constant3/1 -> Relational4/1
  Slice5/1 -> Relational4/2
  win_addr_cnt/1 -> Slice6/1, Slice4/1
  Slice6/1 -> edge_detect1/1(in)
  edge_detect1/1(out) -> Logical1/1
  Slice4/1 -> Delay7/1
  Slice1/1 -> Delay1/1, [current_window]
  Slice2/1 -> edge_detect/1(in)
  Delay7/1 -> Concat1/2
  Concat1/1 -> [rd_addr], rd_addr/1
  Concat2/1 -> rd_timefreq/1, [rd_mcnt]

== system s_b4a4x32kf_nb/sys2/pkt_reord/status0 ==
  out_sync_cnt : Inport
  out_last_missed_ant : Inport  Port=2
  out_missed_err_cnt : Inport  Port=3
  out_timeout_err_cnt : Inport  Port=4
  out_discard_err_cnt : Inport  Port=5
  assert_discard_err_cnt : xbsIndex_r4/Assert  assert_type=on  type_source=Explicitly  gui_display_data_type=Fixed-point  arith_type=Unsigned  n_bits=6  bin_pt=0  preci_type=Single  exp_width=8  frac_width=24  assert_rate=off  rate_source=Explicitly  period=1  output_port=on  block_type=assert
      settings: SourceProductName=The database /home/jmanley/.matlab/R2018a/slblocks_master.db is locked, or a table in the database is locked. (database is locked)
  assert_last_missed_ant : xbsIndex_r4/Assert  assert_type=on  type_source=Explicitly  gui_display_data_type=Fixed-point  arith_type=Unsigned  n_bits=6  bin_pt=0  preci_type=Single  exp_width=8  frac_width=24  assert_rate=off  rate_source=Explicitly  period=1  output_port=on  block_type=assert
      settings: SourceProductName=The database /home/jmanley/.matlab/R2018a/slblocks_master.db is locked, or a table in the database is locked. (database is locked)
  assert_missed_err_cnt : xbsIndex_r4/Assert  assert_type=on  type_source=Explicitly  gui_display_data_type=Fixed-point  arith_type=Unsigned  n_bits=6  bin_pt=0  preci_type=Single  exp_width=8  frac_width=24  assert_rate=off  rate_source=Explicitly  period=1  output_port=on  block_type=assert
      settings: SourceProductName=The database /home/jmanley/.matlab/R2018a/slblocks_master.db is locked, or a table in the database is locked. (database is locked)
  assert_sync_cnt : xbsIndex_r4/Assert  assert_type=on  type_source=Explicitly  gui_display_data_type=Fixed-point  arith_type=Unsigned  n_bits=6  bin_pt=0  preci_type=Single  exp_width=8  frac_width=24  assert_rate=off  rate_source=Explicitly  period=1  output_port=on  block_type=assert
      settings: SourceProductName=The database /home/jmanley/.matlab/R2018a/slblocks_master.db is locked, or a table in the database is locked. (database is locked)
  assert_timeout_err_cnt : xbsIndex_r4/Assert  assert_type=on  type_source=Explicitly  gui_display_data_type=Fixed-point  arith_type=Unsigned  n_bits=6  bin_pt=0  preci_type=Single  exp_width=8  frac_width=24  assert_rate=off  rate_source=Explicitly  period=1  output_port=on  block_type=assert
      settings: SourceProductName=The database /home/jmanley/.matlab/R2018a/slblocks_master.db is locked, or a table in the database is locked. (database is locked)
  cast_gw : xbsIndex_r4/Convert  gui_display_data_type=Fixed-point  arith_type=Unsigned  n_bits=32  bin_pt=0  float_type=Single  exp_bits=8  fraction_bits=24  quantization=Truncate  overflow=Wrap  en=off  latency=1  pipeline=off  dbl_ovrd=off  block_type=convert
      settings: SourceProductName=The database /home/jmanley/.matlab/R2018a/slblocks_master.db is locked, or a table in the database is locked. (database is locked)
  concatenate : xbsIndex_r4/Concat  num_inputs=5  dbl_ovrd=off  block_type=concat
      settings: SourceProductName=The database /home/jmanley/.matlab/R2018a/slblocks_master.db is locked, or a table in the database is locked. (database is locked)
  io_delay : xbsIndex_r4/Delay  rst=off  infoeditControl=Selection of Reset will increase slice count due to use of real FFs and instead of SRLs  en=off  latency=1  reg_retiming=on  dbl_ovrd=off  block_type=delay
      settings: SourceProductName=The database /home/jmanley/.matlab/R2018a/slblocks_master.db is locked, or a table in the database is locked. (database is locked)
  reint{1..5} (5 alike) : xbsIndex_r4/Reinterpret  force_arith_type=on  arith_type=Unsigned  force_bin_pt=on  bin_pt=0  block_type=reinterpret
      settings: SourceProductName=The database /home/jmanley/.matlab/R2018a/slblocks_master.db is locked, or a table in the database is locked. (database is locked)
  s_b4a4x32kf_nb_sys2_pkt_reord_status0_user_data_in : xbsIndex_r4/Gateway Out  inherit_from_input=off  hdl_port=on  rows=1  columns=1  UseAsDAC=off  DACChannel='1'  interface=None  automatic_assignment=on  address_offset=hex2dec('00')  intf_name=''  intf_description=''  timing_constraint=None  locs_specified=off  LOCs={}  io_standard={}  block_type=gatewayout
      settings: SourceProductName=The database /home/jmanley/.matlab/R2018a/slblocks_master.db is locked, or a table in the database is locked. (database is locked)
  sim_out : Terminator
  wires:
  concatenate/1 -> io_delay/1
  io_delay/1 -> cast_gw/1
  cast_gw/1 -> s_b4a4x32kf_nb_sys2_pkt_reord_status0_user_data_in/1
  s_b4a4x32kf_nb_sys2_pkt_reord_status0_user_data_in/1 -> sim_out/1
  out_sync_cnt/1 -> assert_sync_cnt/1
  assert_sync_cnt/1 -> reint1/1
  reint1/1 -> concatenate/1
  out_last_missed_ant/1 -> assert_last_missed_ant/1
  assert_last_missed_ant/1 -> reint2/1
  reint2/1 -> concatenate/2
  out_missed_err_cnt/1 -> assert_missed_err_cnt/1
  assert_missed_err_cnt/1 -> reint3/1
  reint3/1 -> concatenate/3
  out_timeout_err_cnt/1 -> assert_timeout_err_cnt/1
  assert_timeout_err_cnt/1 -> reint4/1
  reint4/1 -> concatenate/4
  out_discard_err_cnt/1 -> assert_discard_err_cnt/1
  assert_discard_err_cnt/1 -> reint5/1
  reint5/1 -> concatenate/5

== system s_b4a4x32kf_nb/sys2/pkt_reord/status1 ==
  out_dv_per_sec : Inport
  assert_dv_per_sec : xbsIndex_r4/Assert  assert_type=on  type_source=Explicitly  gui_display_data_type=Fixed-point  arith_type=Unsigned  n_bits=32  bin_pt=0  preci_type=Single  exp_width=8  frac_width=24  assert_rate=off  rate_source=Explicitly  period=1  output_port=on  block_type=assert
      settings: SourceProductName=The database /home/jmanley/.matlab/R2018a/slblocks_master.db is locked, or a table in the database is locked. (database is locked)
  cast_gw : xbsIndex_r4/Convert  gui_display_data_type=Fixed-point  arith_type=Unsigned  n_bits=32  bin_pt=0  float_type=Single  exp_bits=8  fraction_bits=24  quantization=Truncate  overflow=Wrap  en=off  latency=1  pipeline=off  dbl_ovrd=off  block_type=convert
      settings: SourceProductName=The database /home/jmanley/.matlab/R2018a/slblocks_master.db is locked, or a table in the database is locked. (database is locked)
  io_delay : xbsIndex_r4/Delay  rst=off  infoeditControl=Selection of Reset will increase slice count due to use of real FFs and instead of SRLs  en=off  latency=0  reg_retiming=on  dbl_ovrd=off  block_type=delay
      settings: SourceProductName=The database /home/jmanley/.matlab/R2018a/slblocks_master.db is locked, or a table in the database is locked. (database is locked)
  reint1 : xbsIndex_r4/Reinterpret  force_arith_type=on  arith_type=Unsigned  force_bin_pt=on  bin_pt=0  block_type=reinterpret
      settings: SourceProductName=The database /home/jmanley/.matlab/R2018a/slblocks_master.db is locked, or a table in the database is locked. (database is locked)
  s_b4a4x32kf_nb_sys2_pkt_reord_status1_user_data_in : xbsIndex_r4/Gateway Out  inherit_from_input=off  hdl_port=on  rows=1  columns=1  UseAsDAC=off  DACChannel='1'  interface=None  automatic_assignment=on  address_offset=hex2dec('00')  intf_name=''  intf_description=''  timing_constraint=None  locs_specified=off  LOCs={}  io_standard={}  block_type=gatewayout
      settings: SourceProductName=The database /home/jmanley/.matlab/R2018a/slblocks_master.db is locked, or a table in the database is locked. (database is locked)
  sim_out : Terminator
  wires:
  io_delay/1 -> cast_gw/1
  cast_gw/1 -> s_b4a4x32kf_nb_sys2_pkt_reord_status1_user_data_in/1
  s_b4a4x32kf_nb_sys2_pkt_reord_status1_user_data_in/1 -> sim_out/1
  out_dv_per_sec/1 -> assert_dv_per_sec/1
  assert_dv_per_sec/1 -> reint1/1
  reint1/1 -> io_delay/1

== system s_b4a4x32kf_nb/sys2/pkt_reord/time_freq_unpack ==
  din : Inport
  xeng_id : Inport  Port=2
  Concat2 : xbsIndex_r4/Concat  num_inputs=2  dbl_ovrd=off  block_type=concat
      settings: SourceProductName=The database /home/jmanley/.matlab/R2018a/slblocks_master.db is locked, or a table in the database is locked. (database is locked)
  Slice2 : xbsIndex_r4/Slice  nbits=chan_bits-xeng_bits  boolean_output=off  mode=Lower Bit Location + Width  bit1=-1  base1=MSB of Input  bit0=0  base0=LSB of Input  dbl_ovrd=off  block_type=slice
      settings: SourceProductName=The database /home/jmanley/.matlab/R2018a/slblocks_master.db is locked, or a table in the database is locked. (database is locked)  block_version=10.1.3
  Slice3 : xbsIndex_r4/Slice  nbits=1  boolean_output=off  mode=Two Bit Locations  bit1=0  base1=MSB of Input  bit0=chan_bits-xeng_bits  base0=LSB of Input  dbl_ovrd=off  block_type=slice
      settings: SourceProductName=The database /home/jmanley/.matlab/R2018a/slblocks_master.db is locked, or a table in the database is locked. (database is locked)  block_version=10.1.3
  time : Outport
  freq : Outport  Port=2
  wires:
  xeng_id/1 -> Concat2/1
  Concat2/1 -> freq/1
  Slice2/1 -> Concat2/2
  Slice3/1 -> time/1
  din/1 -> Slice2/1, Slice3/1
